simulink model "controlloH2rob"  (R2024a)
settings: Solver=VariableStepAuto  StartTime=0.0  StopTime=10.0  RelTol=1e-3
values from neighbouring files (symbols this model uses):
  B = {B1, B2, B3, B4}    [HinfLPV_Regulation.m]    (also in L1LPV_Regulation.m; L1_H2_Hinf_dosso.m = [; L1_H2_Hinf_strada_dissestata.m = [; controlloH2H8_H8alfa.m = [)
  C = [1 0 0 0 0 0 0 0 ... (first row only)    [L1_H2_Hinf_dosso.m]    (also in L1_H2_Hinf_strada_dissestata.m; controlloH2H8_H8alfa.m; controlloH2Robusto.m = eye(8); controlloH2_dinamico.m = [)
  D = [ ... (first row only)    [controlloH2H8_H8alfa.m]    (also in controlloH2Robusto.m = zeros(8,4); controlloH2_dinamico.m = zeros(4,2); controlloH8_dinamico.m = zeros(4,2); controlloHinfLPV.m = zeros(8,4))
  E = [ ... (first row only)    [L1_H2_Hinf_dosso.m]    (also in L1_H2_Hinf_strada_dissestata.m; controlloH2H8_H8alfa.m; controlloH2Robusto.m; controlloH2_dinamico.m)
  k_h2 = H2_Regulation(A,B,E,C,D22)    [L1_H2_Hinf_dosso.m]    (also in L1_H2_Hinf_strada_dissestata.m; controlloH2Robusto.m = H2_Regulation(A,B,E,C22,D22); controlloH2_dinamico.m = H2_Regulation(A,B,E,C2,D22))
  k_h2rob = H2Rob_Regulation(A1,A2,A3,A4,B,B,B,B,E,E,E,E,C22,D22)    [controlloH2Robusto.m]
  k_sf_max = 20700    [controlloH2Robusto.m]    (also in controlloHinfLPV.m)
  k_sf_min = 15300    [controlloH2Robusto.m]    (also in controlloHinfLPV.m)
  k_sr_max = 25300    [controlloH2Robusto.m]    (also in controlloHinfLPV.m)
  k_sr_min = 18700    [controlloH2Robusto.m]    (also in controlloHinfLPV.m)
  x0 = zeros(8,1)    [L1_H2_Hinf_dosso.m]    (also in L1_H2_Hinf_strada_dissestata.m; controlloH2H8_H8alfa.m; controlloH2Robusto.m; controlloH2_dinamico.m)
settings Model: Creator=alest  LastModifiedBy=alest

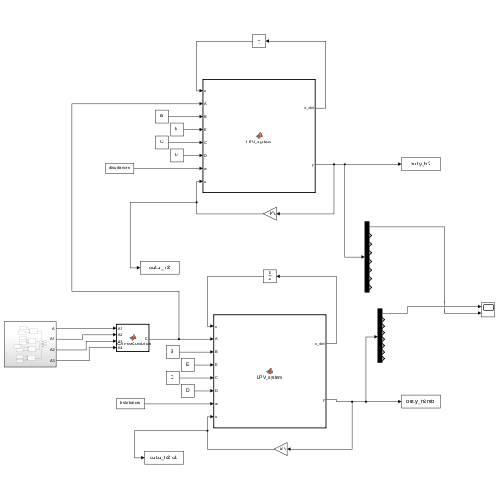
[thumbnail: Simulink's stored preview of the top-level diagram]
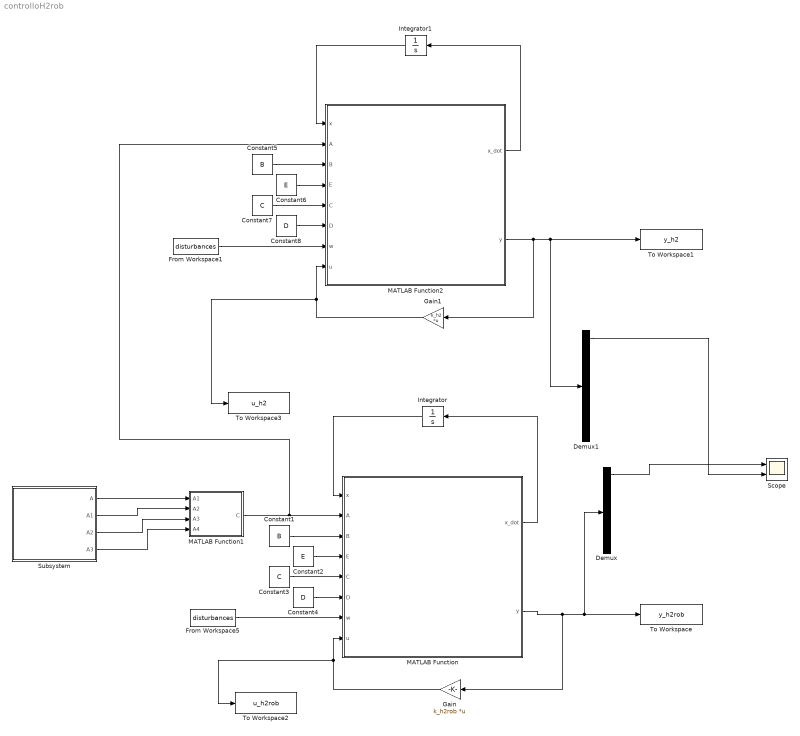
== system controlloH2rob ==
  Constant1 : Constant  Value=B
  Constant2 : Constant  Value=E
  Constant3 : Constant  Value=C
  Constant4 : Constant  Value=D
  Constant5 : Constant  Value=B
  Constant6 : Constant  Value=E
  Constant7 : Constant  Value=C
  Constant8 : Constant  Value=D
  Demux : Demux  Outputs=8
  Demux1 : Demux  Outputs=8
  From Workspace1 : FromWorkspace  VariableName=disturbances
  From Workspace5 : FromWorkspace  VariableName=disturbances
  Gain : Gain  Gain=k_h2rob  Multiplication=Matrix(K*u)
  Gain1 : Gain  Gain=k_h2  Multiplication=Matrix(K*u)
  Integrator : Integrator  InitialCondition=x0
  Integrator1 : Integrator  InitialCondition=x0
  MATLAB Function : MATLAB Function  TreatAsAtomicUnit=on
  MATLAB Function1 : MATLAB Function  TreatAsAtomicUnit=on  SystemSampleTime=0
  MATLAB Function2 : MATLAB Function  TreatAsAtomicUnit=on
  Scope : Scope  NumInputPorts=2
  Subsystem : Subsystem
  To Workspace : ToWorkspace  VariableName=y_h2rob  SaveFormat=Timeseries  SampleTime=-1
  To Workspace1 : ToWorkspace  VariableName=y_h2  SaveFormat=Timeseries  SampleTime=-1
  To Workspace2 : ToWorkspace  VariableName=u_h2rob  SaveFormat=Timeseries  SampleTime=-1
  To Workspace3 : ToWorkspace  VariableName=u_h2  SaveFormat=Timeseries  SampleTime=-1
  wires:
  Constant1/1 -> MATLAB Function/3(B)
  Constant2/1 -> MATLAB Function/4(E)
  Constant3/1 -> MATLAB Function/5(C)
  Constant4/1 -> MATLAB Function/6(D)
  MATLAB Function/2(y) -> Gain/1, Demux/1, To Workspace/1
  Gain/1 -> To Workspace2/1, MATLAB Function/8(u)
  MATLAB Function/1(x_dot) -> Integrator/1
  Integrator/1 -> MATLAB Function/1(x)
  From Workspace5/1 -> MATLAB Function/7(w)
  Subsystem/1(A) -> MATLAB Function1/1(A1)
  Subsystem/2(A1) -> MATLAB Function1/2(A2)
  Subsystem/3(A2) -> MATLAB Function1/3(A3)
  Subsystem/4(A3) -> MATLAB Function1/4(A4)
  MATLAB Function2/2(y) -> Gain1/1, Demux1/1, To Workspace1/1
  Constant7/1 -> MATLAB Function2/5(C)
  Integrator1/1 -> MATLAB Function2/1(x)
  Constant5/1 -> MATLAB Function2/3(B)
  MATLAB Function2/1(x_dot) -> Integrator1/1
  Constant6/1 -> MATLAB Function2/4(E)
  From Workspace1/1 -> MATLAB Function2/7(w)
  Gain1/1 -> To Workspace3/1, MATLAB Function2/8(u)
  Constant8/1 -> MATLAB Function2/6(D)
  MATLAB Function1/1(C) -> MATLAB Function2/2(A), MATLAB Function/2(A)
  Demux1/1 -> Scope/2
  Demux/1 -> Scope/1

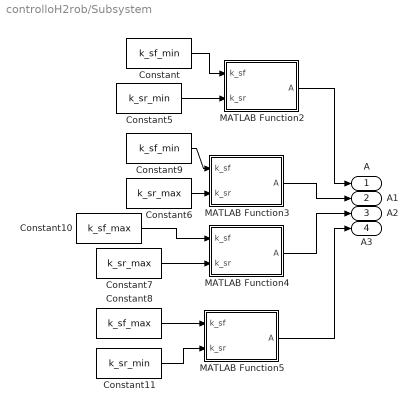
== system controlloH2rob/Subsystem ==
  Constant : Constant  Value=k_sf_min
  Constant10 : Constant  Value=k_sf_max
  Constant11 : Constant  Value=k_sr_min
  Constant5 : Constant  Value=k_sr_min
  Constant6 : Constant  Value=k_sr_max
  Constant7 : Constant  Value=k_sr_max
  Constant8 : Constant  Value=k_sf_max
  Constant9 : Constant  Value=k_sf_min
  MATLAB Function2 : MATLAB Function  TreatAsAtomicUnit=on
  MATLAB Function3 : MATLAB Function  TreatAsAtomicUnit=on
  MATLAB Function4 : MATLAB Function  TreatAsAtomicUnit=on
  MATLAB Function5 : MATLAB Function  TreatAsAtomicUnit=on
  A : Outport
  A1 : Outport  Port=2
  A2 : Outport  Port=3
  A3 : Outport  Port=4
  wires:
  Constant9/1 -> MATLAB Function3/1(k_sf)
  Constant6/1 -> MATLAB Function3/2(k_sr)
  Constant10/1 -> MATLAB Function4/1(k_sf)
  Constant7/1 -> MATLAB Function4/2(k_sr)
  Constant/1 -> MATLAB Function2/1(k_sf)
  MATLAB Function4/1(A) -> A2/1
  Constant5/1 -> MATLAB Function2/2(k_sr)
  Constant11/1 -> MATLAB Function5/2(k_sr)
  Constant8/1 -> MATLAB Function5/1(k_sf)
  MATLAB Function2/1(A) -> A/1
  MATLAB Function3/1(A) -> A1/1
  MATLAB Function5/1(A) -> A3/1

== matlab function controlloH2rob/MATLAB Function1 ==
  data: C output; A1 input; A2 input; A3 input; A4 input
function C = randConvexCombination(A1,A2,A3,A4)
    A={A1,A2,A3,A4};
    % Numero di matrici nella cella
    n = numel(A);

    % Genera pesi casuali
    weights = rand(1, n);

    % Normalizza i pesi affinché la loro somma sia 1
    weights = weights / sum(weights);

    % Dimensione delle matrici (si assume che tutte siano uguali)
    C = zeros(size(A{1}));

    % Calcola la combinazione convessa
    for i = 1:n
        C = C + weights(i) * A{i};
    end

end

== matlab function controlloH2rob/MATLAB Function ==
  data: x_dot output; x input; A input; y output; B input; E input; C input; D input; w input; u input
function [x_dot,y] = LPV_system(x,A,B,E,C,D,w,u)

x_dot=A*x+B*u+E*w;

y = C*x;

end

== matlab function controlloH2rob/Subsystem/MATLAB Function2 ==
  data: k_sf input; A output; k_sr input
function A=calcolaA(k_sf,k_sr)

m_s = 690;    % Massa del corpo principale [kg]
I_psi = 1222;  % Momento d'inerzia rispetto all'asse [kg*m^2]
m_uf = 40;     % Massa della ruota anteriore [kg]
m_ur = 45;     % Massa della ruota posteriore [kg]
k_uf = 200000; % Costante elastica ruota anteriore [N/m]
k_ur = 200000; % Costante elastica ruota posteriore [N/m]
c_sf = 1000;   % Costante smorzamento sospensione anteriore [Ns/m]
c_sr = 1000;   % Costante smorzamento sospensione posteriore [Ns/m]
L_f = 1.3;     % Distanza tra CG e asse anteriore [m]
L_r = 1.5;     % Distanza tra CG e asse posteriore [m]

A = [
    0, 1, 0, 0, 0, 0, 0, 0;
    -(k_sf + k_sr)/m_s, -(c_sf + c_sr)/m_s, (k_sf*L_f - k_sr*L_r)/m_s, (c_sf*L_f - c_sr*L_r)/m_s, k_sf/m_s, c_sf/m_s, k_sr/m_s, c_sr/m_s;
    0, 0, 0, 1, 0, 0, 0, 0;
    (k_sf*L_f - k_sr*L_r)/I_psi, (c_sf*L_f - c_sr*L_r)/I_psi, -(k_sf*L_f^2 + k_sr*L_r^2)/I_psi, -(c_sf*L_f^2 + c_sr*L_r^2)/I_psi, -k_sf*L_f/I_psi, -c_sf*L_f/I_psi, k_sr*L_r/I_psi, c_sr*L_r/I_psi;
    0, 0, 0, 0, 0, 1, 0, 0;
    k_sf/m_uf, c_sf/m_uf, -k_sf*L_f/m_uf, -c_sf*L_f/m_uf, -(k_sf + k_uf)/m_uf, -c_sf/m_uf, 0, 0;
    0, 0, 0, 0, 0, 0, 0, 1;
    k_sr/m_ur, c_sr/m_ur, k_sr*L_r/m_ur, c_sr*L_r/m_ur, 0, 0, -(k_sr + k_ur)/m_ur, -c_sr/m_ur
];

end

== matlab function controlloH2rob/Subsystem/MATLAB Function3 ==
  data: k_sf input; A output; k_sr input
function A=calcolaA(k_sf,k_sr)

m_s = 690;    % Massa del corpo principale [kg]
I_psi = 1222;  % Momento d'inerzia rispetto all'asse [kg*m^2]
m_uf = 40;     % Massa della ruota anteriore [kg]
m_ur = 45;     % Massa della ruota posteriore [kg]
k_uf = 200000; % Costante elastica ruota anteriore [N/m]
k_ur = 200000; % Costante elastica ruota posteriore [N/m]
c_sf = 1000;   % Costante smorzamento sospensione anteriore [Ns/m]
c_sr = 1000;   % Costante smorzamento sospensione posteriore [Ns/m]
L_f = 1.3;     % Distanza tra CG e asse anteriore [m]
L_r = 1.5;     % Distanza tra CG e asse posteriore [m]

A = [
    0, 1, 0, 0, 0, 0, 0, 0;
    -(k_sf + k_sr)/m_s, -(c_sf + c_sr)/m_s, (k_sf*L_f - k_sr*L_r)/m_s, (c_sf*L_f - c_sr*L_r)/m_s, k_sf/m_s, c_sf/m_s, k_sr/m_s, c_sr/m_s;
    0, 0, 0, 1, 0, 0, 0, 0;
    (k_sf*L_f - k_sr*L_r)/I_psi, (c_sf*L_f - c_sr*L_r)/I_psi, -(k_sf*L_f^2 + k_sr*L_r^2)/I_psi, -(c_sf*L_f^2 + c_sr*L_r^2)/I_psi, -k_sf*L_f/I_psi, -c_sf*L_f/I_psi, k_sr*L_r/I_psi, c_sr*L_r/I_psi;
    0, 0, 0, 0, 0, 1, 0, 0;
    k_sf/m_uf, c_sf/m_uf, -k_sf*L_f/m_uf, -c_sf*L_f/m_uf, -(k_sf + k_uf)/m_uf, -c_sf/m_uf, 0, 0;
    0, 0, 0, 0, 0, 0, 0, 1;
    k_sr/m_ur, c_sr/m_ur, k_sr*L_r/m_ur, c_sr*L_r/m_ur, 0, 0, -(k_sr + k_ur)/m_ur, -c_sr/m_ur
];

end

== matlab function controlloH2rob/Subsystem/MATLAB Function4 ==
  data: k_sf input; A output; k_sr input
function A=calcolaA(k_sf,k_sr)

m_s = 690;    % Massa del corpo principale [kg]
I_psi = 1222;  % Momento d'inerzia rispetto all'asse [kg*m^2]
m_uf = 40;     % Massa della ruota anteriore [kg]
m_ur = 45;     % Massa della ruota posteriore [kg]
k_uf = 200000; % Costante elastica ruota anteriore [N/m]
k_ur = 200000; % Costante elastica ruota posteriore [N/m]
c_sf = 1000;   % Costante smorzamento sospensione anteriore [Ns/m]
c_sr = 1000;   % Costante smorzamento sospensione posteriore [Ns/m]
L_f = 1.3;     % Distanza tra CG e asse anteriore [m]
L_r = 1.5;     % Distanza tra CG e asse posteriore [m]

A = [
    0, 1, 0, 0, 0, 0, 0, 0;
    -(k_sf + k_sr)/m_s, -(c_sf + c_sr)/m_s, (k_sf*L_f - k_sr*L_r)/m_s, (c_sf*L_f - c_sr*L_r)/m_s, k_sf/m_s, c_sf/m_s, k_sr/m_s, c_sr/m_s;
    0, 0, 0, 1, 0, 0, 0, 0;
    (k_sf*L_f - k_sr*L_r)/I_psi, (c_sf*L_f - c_sr*L_r)/I_psi, -(k_sf*L_f^2 + k_sr*L_r^2)/I_psi, -(c_sf*L_f^2 + c_sr*L_r^2)/I_psi, -k_sf*L_f/I_psi, -c_sf*L_f/I_psi, k_sr*L_r/I_psi, c_sr*L_r/I_psi;
    0, 0, 0, 0, 0, 1, 0, 0;
    k_sf/m_uf, c_sf/m_uf, -k_sf*L_f/m_uf, -c_sf*L_f/m_uf, -(k_sf + k_uf)/m_uf, -c_sf/m_uf, 0, 0;
    0, 0, 0, 0, 0, 0, 0, 1;
    k_sr/m_ur, c_sr/m_ur, k_sr*L_r/m_ur, c_sr*L_r/m_ur, 0, 0, -(k_sr + k_ur)/m_ur, -c_sr/m_ur
];

end

== matlab function controlloH2rob/Subsystem/MATLAB Function5 ==
  data: k_sf input; A output; k_sr input
function A=calcolaA(k_sf,k_sr)

m_s = 690;    % Massa del corpo principale [kg]
I_psi = 1222;  % Momento d'inerzia rispetto all'asse [kg*m^2]
m_uf = 40;     % Massa della ruota anteriore [kg]
m_ur = 45;     % Massa della ruota posteriore [kg]
k_uf = 200000; % Costante elastica ruota anteriore [N/m]
k_ur = 200000; % Costante elastica ruota posteriore [N/m]
c_sf = 1000;   % Costante smorzamento sospensione anteriore [Ns/m]
c_sr = 1000;   % Costante smorzamento sospensione posteriore [Ns/m]
L_f = 1.3;     % Distanza tra CG e asse anteriore [m]
L_r = 1.5;     % Distanza tra CG e asse posteriore [m]

A = [
    0, 1, 0, 0, 0, 0, 0, 0;
    -(k_sf + k_sr)/m_s, -(c_sf + c_sr)/m_s, (k_sf*L_f - k_sr*L_r)/m_s, (c_sf*L_f - c_sr*L_r)/m_s, k_sf/m_s, c_sf/m_s, k_sr/m_s, c_sr/m_s;
    0, 0, 0, 1, 0, 0, 0, 0;
    (k_sf*L_f - k_sr*L_r)/I_psi, (c_sf*L_f - c_sr*L_r)/I_psi, -(k_sf*L_f^2 + k_sr*L_r^2)/I_psi, -(c_sf*L_f^2 + c_sr*L_r^2)/I_psi, -k_sf*L_f/I_psi, -c_sf*L_f/I_psi, k_sr*L_r/I_psi, c_sr*L_r/I_psi;
    0, 0, 0, 0, 0, 1, 0, 0;
    k_sf/m_uf, c_sf/m_uf, -k_sf*L_f/m_uf, -c_sf*L_f/m_uf, -(k_sf + k_uf)/m_uf, -c_sf/m_uf, 0, 0;
    0, 0, 0, 0, 0, 0, 0, 1;
    k_sr/m_ur, c_sr/m_ur, k_sr*L_r/m_ur, c_sr*L_r/m_ur, 0, 0, -(k_sr + k_ur)/m_ur, -c_sr/m_ur
];

end

== matlab function controlloH2rob/MATLAB Function2 ==
  data: x_dot output; x input; A input; y output; B input; E input; C input; D input; w input; u input
function [x_dot,y] = LPV_system(x,A,B,E,C,D,w,u)

x_dot=A*x+B*u+E*w;

y = C*x;

end
